simulink model "KINvasion"  (Simulink 7.5)
settings: Solver=ode4  SolverMode=SingleTasking  StartTime=0.0  StopTime=inf  FixedStep=0.0005  RelTol=1e-3
StartFcn:
  |  warndlg('Dexterit-E models cannot run under simulation. Please compile your model and run it from within Dexterit-E.');set_param(gcs,'SimulationCommand','stop')
undefined symbols (not defined in the file or in its folder): Process_Video_CMD, Video
libraries: xpclib x5, General x3, KINARM_general x1, KINARM_EP_loads x1
(part 3 of 3)

== matlab function Process_Video_CMD/PVC_core/Embedded MATLAB Function ==
  settings: fimath=|
      | fimath(...
      | 'RoundMode', 'floor',...
      | 'OverflowMode', 'wrap',...
      | 'ProductMode', 'KeepLSB', 'ProductWordLength', 32,...
      | 'SumMode', 'KeepLSB', 'SumWordLength', 32,...
      | 'CastBeforeSum', false)
  data: VCODE input double; vis_cmd_out output double; vis_cmd_cropped output double; frame_sent_trigger output double; frame_number output double; num_used_VCODEs input double
function [vis_cmd_out, vis_cmd_cropped, frame_sent_trigger, frame_number] = fcn(VCODE, num_used_VCODEs)

% Increment a counter on each execution, which corresponds to one increment per packet. This counter is used 
% as a tracking number / "timestamp". Video command acknowledgements refer to this counter.
persistent frame_count
persistent frame_trigger

% maximum size of the vis_cmd_length is limited to 2 MTUs to avoid swamping the UDP system.  Each MTU is ~1500, but
% there is header info in there, so we need to limit total to 2900 bytes.
max_vis_cmd_length = round(2900 / 4);		% vis_cmd is composed of int32, which are 4 bytes each
% max_vis_cmd_length = round(100 / 4);		% FOR TESTING ONLY - Should limit the output to ~2 VCODEs.

if isempty(frame_count)
   frame_count = uint32(0);
end

frame_count = frame_count + 1;
frame_number = frame_count;

if isempty(frame_trigger)
    frame_trigger = 1;
else
    frame_trigger = mod(frame_trigger + 1, 2);
end

frame_sent_trigger = frame_trigger;

% vis_cmd must be a fixed length, so it is initialized to the maximum possible length required.
%  (number of VCODEs * max_single_vis_cmd_length) + 3 int32 for message header, frame count, and "end-of-command" marker
%
% Note: max_single_vis_cmd_length refers to the maximum possible length of a single target (i.e. the number of int32 elements 
% required to define it) within the vis_cmd vector. Currently a triangle with a label is potentially the longest, with
% the following elements (each an int32):
%   1: target type + target on/off status 
%   2: x position
%   3: y position
%   4: fill colour
%   5: stroke colour
%   6: stroke width
%   7: opacity
%   8: base width
%   9: height
%  10: peak offset
%  11: rotation
%  12-24:  maximum length label (up to 50 characters, 4 1-byte characters per int32, with one byte for a null terminator)
%  25: label colour
%  26: label height
%  27: target id when in background

max_single_vis_cmd_length = 27;
num_VCODEs = size(VCODE, 1);
vis_cmd = cast(zeros(max_single_vis_cmd_length * num_VCODEs + 3, 1), 'int32');

index = 1;  % index into vis_cmd

% Create a 4-byte message header.
%   byte 1: version
%     0x20 = Version 2.0
%     0x23 = Version 2.3
%       etc.
%   bytes 2-4: currently unused
header = bitshift(cast(23, 'uint32'), 24);
vis_cmd(index) = cast_int32(header);
index = index + 1;

% Insert the timestamp for this video frame.
vis_cmd(index) = cast_int32(frame_count);
index = index + 1;

% Create target commands from VCODEs.
%
% Note: Because all values are communicated via UDP as int32, distances and orientations are converted from (m) and (rad).
%   - in Dexterit-E 2.0 and later, these values are converted to from (m) to (um) and from (rad) to (urad)
%   - in KINARM-UI 1.4, these values were are converted from (m) to (10 * um) and from (rad) to (degrees)
last_ok_index = 1;		% initialize
for i = 1:num_used_VCODEs

    % #1: Add information common to all targets.
    add_target_id = 0;

    if VCODE(i, 1) == 0  % don't include anything for targets with type 0, i.e. VCODEs that have not been set properly
        continue;
    end
    
    % Target type and on/off status are packed into one int32. The two high bytes are used for the type,
    % and the two low bytes are used for the status.
    status = bitshift(cast(VCODE(i, 1), 'uint32'), 16) + VCODE(i, 2);
    vis_cmd(index) = cast_int32(status);

    vis_cmd(index + 1) = VCODE(i, 3) * 1000000;  % target x position (convert from (m) in VCODE to (um))
    vis_cmd(index + 2) = VCODE(i, 4) * 1000000;  % target y position (convert from (m) in VCODE to (um))

	vis_cmd(index + 3) = cast_int32(VCODE(i, 5));  % fill colour
	vis_cmd(index + 4) = cast_int32(VCODE(i, 6));  % stroke colour

    vis_cmd(index + 5) = VCODE(i, 7) * 1000000;  % stroke width (convert from (m) in VCODE to (um))
    
    vis_cmd(index + 6) = VCODE(i, 9);  % opacity

    % #2: Add target type-specific information.
    target_type = VCODE(i, 1);
    
    if target_type >= 100
        add_target_id = 1;
        target_type = target_type - 100;
    end

    if target_type == 1 || target_type == 11
        
        % Handle circle target:
        vis_cmd(index + 7) = VCODE(i, 10) * 1000000;  % radius (convert from (m) in VCODE to (um))

        index = index + 8;

    elseif target_type == 2 || target_type == 12

        % Handle ellipse target:
        vis_cmd(index + 7) = VCODE(i, 10) * 1000000;  % major radius (convert from (m) in VCODE to (um))
        vis_cmd(index + 8) = VCODE(i, 11) * 1000000;  % minor radius (convert from (m) in VCODE to (um))
        vis_cmd(index + 9) = VCODE(i, 12) * 1000000;  % orientation (convert from (rad) in VCODE to (urad))

        index = index + 10;

    elseif target_type == 3 || target_type == 13

        % Handle rectangle target:
        vis_cmd(index + 7) = VCODE(i, 10) * 1000000;  % length (convert from (m) in VCODE to (um))
        vis_cmd(index + 8) = VCODE(i, 11) * 1000000;  % height (convert from (m) in VCODE to (um))
        vis_cmd(index + 9) = VCODE(i, 12) * 1000000;  % orientation (convert from (rad) in VCODE to (um))

        index = index + 10;

    elseif target_type == 4 || target_type == 14

        % Handle line target:
        vis_cmd(index + 7) = VCODE(i, 10) * 1000000;  % endpoint x position, relative to start point (convert from (m) in VCODE to (um))
        vis_cmd(index + 8) = VCODE(i, 11) * 1000000;  % endpoint y position, relative to start point (convert from (m) in VCODE to (um))

        index = index + 9;

    elseif target_type == 5 || target_type == 15

        % Handle triangle target:
        vis_cmd(index + 7) = VCODE(i, 10) * 1000000;  % base width (convert from (m) in VCODE to (um))
        vis_cmd(index + 8) = VCODE(i, 11) * 1000000;  % height (convert from (m) in VCODE to (um))
        vis_cmd(index + 9) = VCODE(i, 12) * 1000000;  % peak offset (convert from (m) in VCODE to (um))
        vis_cmd(index + 10) = VCODE(i, 13) * 1000000;  % orientation (convert from (rad) in VCODE to (urad))

        index = index + 11;

    else
        index = index + 7;
    end
    
    % #3: Add the label information (if the target is of a labelled type).
    if (target_type >= 11 && target_type <= 15) || (target_type >= 111 && target_type <= 115)
        j = 0;
        
        while j < 13
            c1 = cast(VCODE(i, 15 + j * 4), 'uint32');
            c2 = cast(VCODE(i, 15 + j * 4 + 1), 'uint32');
            
            if j < 12
                c3 = cast(VCODE(i, 15 + j * 4 + 2), 'uint32');
                c4 = cast(VCODE(i, 15 + j * 4 + 3), 'uint32');
            else
                c3 = uint32(0);
                c4 = uint32(0);
            end

            vis_cmd(index + j) = bitshift(c1, 24) + bitshift(c2, 16) + bitshift(c3, 8) + c4;
            
            if c1 == 0 || c2 == 0 || c3 == 0 || c4 == 0
                break;
            end
            
            j = j + 1;
        end
        
        j = j + 1;
        
        vis_cmd(index + j) = cast_int32(VCODE(i, 65));    % label colour
        vis_cmd(index + j + 1) = VCODE(i, 66) * 1000000;  % label height (convert from (m) in VCODE to (um))
        
        index = index + j + 2;
    end
    
    % #4: Add the target ID if the target is being placed in the background.
	if add_target_id > 0
        vis_cmd(index) = cast_int32(VCODE(i, 8));
        index = index + 1;
	end
	
	% if the current index < max_vis_cmd_length, then the VCODEs just added will fit in the vis_cmd_out 
	if index < max_vis_cmd_length
		last_ok_index = index;
	end
end

% only output full VCODEs so as to not confuse DexDisplay
vis_cmd_out = cast(zeros(max_vis_cmd_length, 1), 'int32');
for ii = 1:(last_ok_index - 1)
	vis_cmd_out(ii) = vis_cmd(ii);
end

if last_ok_index == index
	vis_cmd_cropped = 0;
else
	vis_cmd_cropped = 1;
end

% Set the "end-of-command" marker: 0xFFFF0000 instead of a target type indicates end of target commands within the vis_cmd vector.
vis_cmd_out(last_ok_index) = cast_int32(bitshift(cast(65535, 'uint32'), 16));
				
% The typecast function is not yet available for Embedded Matlab. This function implements a cast from uint32 to int32.
function output_int32 = cast_int32(input_uint32)

if input_uint32 > 2^31
	temp = cast(input_uint32 - 2^31, 'int32');	% remove MSB and cast to int32
	output_int32 = temp - 2^30 - 2^30;			% subtract 2^31 (because 2^31 is not int32, subtract 2^30 twice)
else
	output_int32 = cast(input_uint32, 'int32');
end

== stateflow chart Process_Video_CMD/PVC_core/Latency Tracking Machine ==
  state A/
    average_ack_delay = total_ack_delay / max(total_acks, 1);
  note: Two indexes into the array of frame numbers (and also that of timestamps) are kept: i and j. The former is always the index of the frame number most
      | recently stored in the array (i.e. the number of the frame most recently sent out), while the latter is used to iterate over the array.
      |
      | When an acknowledged frame number is received, the chart's outputs are updated and the index of that frame in the array is stored so that it cannot be
      | "acknowledged" again. Searches for subsequent frame numbers begin at one beyond that index, and continue only up to the most recent unacknowledged
      | number. If an acknowledgement for a number that is not in the array is received (i.e. either a legitimate but late acknowledgement, for which the frame
      | number has already been cycled out of the array, or an illegitimate / erroneous acknowledgement) the chart's outputs are not changed.
  (default) -> (junction 97) : { j = 0; }
  A -> (junction 99) [order 1] : e_clock
      | { clock_count = clock_count + 1; }
  A -> A [order 2] : e_frame_sent/
      | i = uint32(fmod(i + 1, 500));
      | sent_frame_numbers[i] = frame_number;
      | last_frame_sent = frame_number;
      | sent_times[i] = clock_count;
  (junction 91) -> (junction 92) [order 1] : [has_received_ack > 0]
      | { j = last_ack_position + 1; }
  (junction 91) -> A [order 2]
  (junction 92) -> (junction 93)
  (junction 93) -> (junction 92) [order 1] : [sent_frame_numbers[j] != ack_number && j != i]
      | { j = uint32(fmod(double(j + 1), 500.0)); }
  (junction 93) -> (junction 94) [order 2] : [sent_frame_numbers[j] == ack_number]
      | {
      |   total_acks = total_acks + 1;
      |   total_ack_delay = total_ack_delay + clock_count - sent_times[j];
      |
      |   last_frame_acknowledged = ack_number;
      |   last_frame_ack_delay = clock_count - sent_times[j];
      |
      |   last_ack_position = j;
      | }
  (junction 93) -> (junction 95) [order 3]
  (junction 95) -> (junction 96)
  (junction 96) -> A
  (junction 97) -> (junction 98)
  (junction 98) -> (junction 97) [order 1] : [ j < 500 ]
      | {
      |   sent_frame_numbers[j] = -1;
      |   sent_times[j] = -1;
      |   j = j + 1;
      | }
  (junction 98) -> A [order 2]
  (junction 99) -> (junction 91)
  data: clock_count local double =0; sent_times local double size=500; sent_frame_numbers local uint32 size=500; i local uint32 =0; frame_number input uint32; ack_number input uint32; has_received_ack input double; total_ack_delay local double =0.0; total_acks local double =0; average_ack_delay output double =-1; last_frame_sent output double =-1; j local uint32 =0; last_ack_position local uint32 =0; last_frame_acknowledged output double =-1; last_frame_ack_delay output double =-1
  events: e_clock input RISING_EDGE_EVENT; e_frame_sent input EITHER_EDGE_EVENT
